simulink model "fft_biplex_real_4x_dsp48_opt_test"  (Simulink 7.4)
settings: Solver=VariableStepDiscrete  StartTime=0.0  StopTime=128  RelTol=1e-3
libraries: xbsIndex_r4 x620, casper_library_misc x24, casper_library_delays x6, casper_library_ffts_twiddle x1, simulink x1
(part 5 of 7)

== system fft_biplex_real_4x_dsp48_opt_test/fft_biplex_real_4x/biplex_core/fft_stage_3/butterfly_direct ==
  a : Inport  OutDataType=sfix(16)  OutScaling=2^0
  b : Inport  Port=2  OutDataType=sfix(16)  OutScaling=2^0
  sync : Inport  Port=3  OutDataType=sfix(16)  OutScaling=2^0
  shift : Inport  Port=4  OutDataType=sfix(16)  OutScaling=2^0
  Logical : xbsIndex_r4/Logical  logical_function=OR  inputs=4  en=off  latency=0  precision=Full  arith_type=Unsigned  n_bits=16  bin_pt=0  align_bp=on  dbl_ovrd=off  block_type=logical
      settings: block_version=11.4
  Mux{0..3} (4 alike) : xbsIndex_r4/Mux  inputs=2  en=off  latency=1  precision=Full  arith_type=Unsigned  n_bits=16  bin_pt=14  quantization=Truncate  overflow=Wrap  dbl_ovrd=off  block_type=mux
      settings: block_version=11.4
  Scale{0..3} (4 alike) : xbsIndex_r4/Scale  scale_factor=-1  dbl_ovrd=off  block_type=scale
  cadd : Subsystem  AncestorBlock=casper_library_misc/caddsub_dsp48e  mask(caddsub_dsp48e){mode=Addition, n_bits_a=8, bin_pt_a=7, n_bits_b=12, bin_pt_b=9, full_precision=on, n_bits_c=19, bin_pt_c=17, quantization=Truncate, overflow=Wrap, cast_latency=0}
      mask prompts: mode "Operation:"; n_bits_a "Bit width 'a':"; bin_pt_a "Binary point 'a':"; n_bits_b "Bit width 'b':"; bin_pt_b "Binary point 'b':"; full_precision "Full precision"; n_bits_c "Bit width out:"; bin_pt_c "Binary point out:"; cast_latency "Cast Latency:"
      mask help:
      | Adds or subtracts two complex numbers using a DSP48E.
      |
      | The two inputs can have different bit widths and binary points, but their sum cannot exceed 24 bits.
      mask init: same as fft_biplex_real_4x_dsp48_opt_test/fft_biplex_real_4x/bi_real_unscr_4x/hilbert_dsp48e0/cadd
      settings: AttributesFormatString=|
      | 8_7 + 12_9 ==> 13_9
      | Mode=Addition
      | Latency=2
      mask StyleString: popup(Addition|Subtraction),edit,edit,edit,edit,checkbox,edit,edit,popup(Truncate|Round  (unbiased: +/- Inf)|Round  (unbiased: Even Values)),popup(Wrap|Saturate|Flag as error),edit
      mask CallbackString:
      | |||||thisVariable = 'full_precision';
      | affectedVars = { ...
      |     'n_bits_c', ...
      |     'bin_pt_c', ...
      |     'quantization', ...
      |     'overflow', ...
      |     'cast_latency', ...
      | };
      | 
      | thisBlock = gcb();
      | thisVarState = get_param(thisBlock, thisVariable);
      | maskNames = get_param(thisBlock, 'MaskNames');
      | maskEnables = get_param(thisBlock, 'MaskEnables');
      | 
      | if strcmp(thisVarState, 'on'),
      |     targVarState = 'off';
      | else,
      |     targVarState = 'on';
      | end
      | 
      | for varName = affectedVars
      |     varIndex = find(ismember(maskNames, varName));
      |     maskEnables{varIndex} = targVarState;
      | end
      | 
      | set_param(thisBlock, 'MaskEnables', maskEnables);|||||
      mask TabNameString: Basic,Basic,Basic,Basic,Basic,Output Type,Output Type,Output Type,Output Type,Output Type,Output Type
  convert_of0 : Subsystem  AncestorBlock=casper_library_misc/convert_of  mask(convert_of){bit_width_i=14, binary_point_i=10, bit_width_o=8, binary_point_o=7, latency=1, overflow=Wrap, quantization=Truncate}
      mask prompts: bit_width_i "Bit Width In"; binary_point_i "Binary Point In"; bit_width_o "Bit Width Out"; binary_point_o "Binary Point Out"; overflow "Overflow Behaviour"; quantization "Quantization Behaviour"
      mask help:
      | Converts from one 2's complement bit-width
      | and/or binary point position to another.
      | Includes underflow/overflow indicator.
      mask init: same as fft_biplex_real_4x_dsp48_opt_test/fft_biplex_real_4x/biplex_core/fft_stage_1/butterfly_direct/convert_of0
      settings: AttributesFormatString=[14,10]->[8,7]
      mask StyleString: edit,edit,edit,edit,edit,popup(Wrap|Saturate|Error),popup(Truncate|Round  (unbiased: +/- Inf)|Round  (unbiased: even values))
  convert_of1 : Subsystem  AncestorBlock=casper_library_misc/convert_of  mask(convert_of){bit_width_i=14, binary_point_i=10, bit_width_o=8, binary_point_o=7, latency=1, overflow=Wrap, quantization=Truncate}
      mask prompts: bit_width_i "Bit Width In"; binary_point_i "Binary Point In"; bit_width_o "Bit Width Out"; binary_point_o "Binary Point Out"; overflow "Overflow Behaviour"; quantization "Quantization Behaviour"
      mask help:
      | Converts from one 2's complement bit-width
      | and/or binary point position to another.
      | Includes underflow/overflow indicator.
      mask init: same as fft_biplex_real_4x_dsp48_opt_test/fft_biplex_real_4x/biplex_core/fft_stage_1/butterfly_direct/convert_of0
      settings: AttributesFormatString=[14,10]->[8,7]
      mask StyleString: edit,edit,edit,edit,edit,popup(Wrap|Saturate|Error),popup(Truncate|Round  (unbiased: +/- Inf)|Round  (unbiased: even values))
  convert_of2 : Subsystem  AncestorBlock=casper_library_misc/convert_of  mask(convert_of){bit_width_i=14, binary_point_i=10, bit_width_o=8, binary_point_o=7, latency=1, overflow=Wrap, quantization=Truncate}
      mask prompts: bit_width_i "Bit Width In"; binary_point_i "Binary Point In"; bit_width_o "Bit Width Out"; binary_point_o "Binary Point Out"; overflow "Overflow Behaviour"; quantization "Quantization Behaviour"
      mask help:
      | Converts from one 2's complement bit-width
      | and/or binary point position to another.
      | Includes underflow/overflow indicator.
      mask init: same as fft_biplex_real_4x_dsp48_opt_test/fft_biplex_real_4x/biplex_core/fft_stage_1/butterfly_direct/convert_of0
      settings: AttributesFormatString=[14,10]->[8,7]
      mask StyleString: edit,edit,edit,edit,edit,popup(Wrap|Saturate|Error),popup(Truncate|Round  (unbiased: +/- Inf)|Round  (unbiased: even values))
  convert_of3 : Subsystem  AncestorBlock=casper_library_misc/convert_of  mask(convert_of){bit_width_i=14, binary_point_i=10, bit_width_o=8, binary_point_o=7, latency=1, overflow=Wrap, quantization=Truncate}
      mask prompts: bit_width_i "Bit Width In"; binary_point_i "Binary Point In"; bit_width_o "Bit Width Out"; binary_point_o "Binary Point Out"; overflow "Overflow Behaviour"; quantization "Quantization Behaviour"
      mask help:
      | Converts from one 2's complement bit-width
      | and/or binary point position to another.
      | Includes underflow/overflow indicator.
      mask init: same as fft_biplex_real_4x_dsp48_opt_test/fft_biplex_real_4x/biplex_core/fft_stage_1/butterfly_direct/convert_of0
      settings: AttributesFormatString=[14,10]->[8,7]
      mask StyleString: edit,edit,edit,edit,edit,popup(Wrap|Saturate|Error),popup(Truncate|Round  (unbiased: +/- Inf)|Round  (unbiased: even values))
  csub : Subsystem  AncestorBlock=casper_library_misc/caddsub_dsp48e  mask(caddsub_dsp48e){mode=Subtraction, n_bits_a=8, bin_pt_a=7, n_bits_b=12, bin_pt_b=9, full_precision=on, n_bits_c=19, bin_pt_c=17, quantization=Truncate, overflow=Wrap, cast_latency=0}
      mask prompts: mode "Operation:"; n_bits_a "Bit width 'a':"; bin_pt_a "Binary point 'a':"; n_bits_b "Bit width 'b':"; bin_pt_b "Binary point 'b':"; full_precision "Full precision"; n_bits_c "Bit width out:"; bin_pt_c "Binary point out:"; cast_latency "Cast Latency:"
      mask help:
      | Adds or subtracts two complex numbers using a DSP48E.
      |
      | The two inputs can have different bit widths and binary points, but their sum cannot exceed 24 bits.
      mask init: same as fft_biplex_real_4x_dsp48_opt_test/fft_biplex_real_4x/bi_real_unscr_4x/hilbert_dsp48e0/cadd
      settings: AttributesFormatString=|
      | 8_7 + 12_9 ==> 13_9
      | Mode=Subtraction
      | Latency=2
      mask StyleString: popup(Addition|Subtraction),edit,edit,edit,edit,checkbox,edit,edit,popup(Truncate|Round  (unbiased: +/- Inf)|Round  (unbiased: Even Values)),popup(Wrap|Saturate|Flag as error),edit
      mask CallbackString:
      | |||||thisVariable = 'full_precision';
      | affectedVars = { ...
      |     'n_bits_c', ...
      |     'bin_pt_c', ...
      |     'quantization', ...
      |     'overflow', ...
      |     'cast_latency', ...
      | };
      | 
      | thisBlock = gcb();
      | thisVarState = get_param(thisBlock, thisVariable);
      | maskNames = get_param(thisBlock, 'MaskNames');
      | maskEnables = get_param(thisBlock, 'MaskEnables');
      | 
      | if strcmp(thisVarState, 'on'),
      |     targVarState = 'off';
      | else,
      |     targVarState = 'on';
      | end
      | 
      | for varName = affectedVars
      |     varIndex = find(ismember(maskNames, varName));
      |     maskEnables{varIndex} = targVarState;
      | end
      | 
      | set_param(thisBlock, 'MaskEnables', maskEnables);|||||
      mask TabNameString: Basic,Basic,Basic,Basic,Basic,Output Type,Output Type,Output Type,Output Type,Output Type,Output Type
  ri_to_c01 : casper_library_misc/ri_to_c  SystemSampleTime=-1
  ri_to_c23 : casper_library_misc/ri_to_c  SystemSampleTime=-1
  shift_delay : xbsIndex_r4/Delay  en=off  latency=2  dbl_ovrd=off  reg_retiming=off  block_type=delay
      settings: block_version=11.4
  sync_delay : xbsIndex_r4/Delay  en=off  latency=4  dbl_ovrd=off  reg_retiming=on  block_type=delay
      settings: block_version=11.4
  twiddle_general_4mult : Subsystem  AncestorBlock=casper_library_ffts_twiddle/twiddle_general_4mult  mask(twiddle_general_4mult){Coeffs=getfield( getfield( get_param( gcb,'UserData' ), 'parameters'),'Coeffs'), StepPeriod=0, coeffs_bram=off, coeff_bit_width=8, input_bit_width=8, add_latency=2, mult_latency=3, bram_latency=1, conv_latency=1, arch=Virtex5, use_hdl=on, use_embedded=off, quantization=Truncate, overflow=Wrap}
      mask prompts: Coeffs "Coefficients:"; StepPeriod "Coefficient Step Period (2^?)"; coeffs_bram "Store coefficients in BRAM"; coeff_bit_width "Coefficient Bit Width"; input_bit_width "Input Bit Width"; add_latency "Add Latency"; mult_latency "Mult Latency"; bram_latency "BRAM Latency"; conv_latency "Convert Latency"; arch "Architecture"; use_hdl "Use behavioural HDL for multipliers"; use_embedded "Use embedded multipliers"; quantization "Quantization Behavior"; overflow "Overflow Behavior"
      mask help:
      | Used in biplex pipelined FFT. Implements
      | (a+bi)(c+di) as (ac-bd)+i(ad+bc) with four
      | multipliers
      mask init:
      | twiddle_general_4mult_init(gcb, ...
      |     'Coeffs', Coeffs, ...
      |     'StepPeriod', StepPeriod, ...
      |     'coeffs_bram', coeffs_bram, ...
      |     'coeff_bit_width', coeff_bit_width, ...
      |     'input_bit_width', input_bit_width, ...
      |     'add_latency', add_latency, ...
      |     'mult_latency', mult_latency, ...
      |     'bram_latency', bram_latency, ...
      |     'conv_latency', conv_latency, ...
      |     'arch', arch, ...
      |     'use_hdl', use_hdl, ...
      |     'use_embedded', use_embedded, ...
      |     'quantization', quantization, ...
      |     'overflow', overflow)
      settings: AttributesFormatString=|
      | data=(8,7)
      | coeffs=(8,6)
      | Virtex5
      | (Truncate,Wrap)
      mask StyleString: edit,edit,checkbox,edit,edit,edit,edit,edit,edit,popup(Virtex2Pro|Virtex5),checkbox,checkbox,popup(Truncate|Round  (unbiased: +/- Inf)|Round  (unbiased: Even Values)),popup(Wrap|Saturate|Error)
      mask CallbackString:
      | ||||||||||use_hdl = get_param(gcb,'use_hdl');
      | visibs = get_param(gcb, 'MaskVisibilities');
      | if( strcmp(use_hdl,'on')),
      |     set_param(gcb, 'use_embedded','off');
      |     visibs{12} = 'off';
      | else,
      |     visibs{12} = 'on';
      | end
      | set_param(gcb, 'MaskVisibilities', visibs);|||
  a+bw : Outport  OutDataType=sfix(16)  OutScaling=2^0
  a-bw : Outport  Port=2  OutDataType=sfix(16)  OutScaling=2^0
  of : Outport  Port=3  OutDataType=sfix(16)  OutScaling=2^0
  sync_out : Outport  Port=4
  wires:
  a/1 -> twiddle_general_4mult/1(a)
  b/1 -> twiddle_general_4mult/2(b)
  sync/1 -> twiddle_general_4mult/3(sync)
  twiddle_general_4mult/1(a_re) -> cadd/1(a_re), csub/1(a_re)
  twiddle_general_4mult/2(a_im) -> cadd/2(a_im), csub/2(a_im)
  twiddle_general_4mult/3(bw_re) -> cadd/3(b_re), csub/3(b_re)
  twiddle_general_4mult/4(bw_im) -> cadd/4(b_im), csub/4(b_im)
  twiddle_general_4mult/5(sync_out) -> sync_delay/1
  shift/1 -> shift_delay/1
  shift_delay/1 -> Mux0/1, Mux1/1, Mux2/1, Mux3/1
  cadd/1(c_re) -> Mux0/2, Scale0/1
  cadd/2(c_im) -> Mux1/2, Scale1/1
  csub/1(c_re) -> Mux2/2, Scale2/1
  csub/2(c_im) -> Mux3/2, Scale3/1
  Scale0/1 -> Mux0/3
  Scale1/1 -> Mux1/3
  Scale2/1 -> Mux2/3
  Scale3/1 -> Mux3/3
  Mux0/1 -> convert_of0/1(din)
  Mux1/1 -> convert_of1/1(din)
  Mux2/1 -> convert_of2/1(din)
  Mux3/1 -> convert_of3/1(din)
  convert_of0/1(dout) -> ri_to_c01/1
  convert_of1/1(dout) -> ri_to_c01/2
  convert_of2/1(dout) -> ri_to_c23/1
  convert_of3/1(dout) -> ri_to_c23/2
  convert_of0/2(of) -> Logical/1
  convert_of1/2(of) -> Logical/2
  convert_of2/2(of) -> Logical/3
  convert_of3/2(of) -> Logical/4
  ri_to_c01/1 -> a+bw/1
  ri_to_c23/1 -> a-bw/1
  Logical/1 -> of/1
  sync_delay/1 -> sync_out/1

== system fft_biplex_real_4x_dsp48_opt_test/fft_biplex_real_4x/biplex_core/fft_stage_3/delay_b ==
  In1 : Inport  OutDataType=sfix(16)  OutScaling=2^0
  delay_slr : xbsIndex_r4/Delay  en=off  latency=DelayLen  dbl_ovrd=off  reg_retiming=off  block_type=delay
      settings: xl_area=[0, 0, 0, 0, 0, 0, 0]  block_version=9.1.01
  Out1 : Outport  OutDataType=sfix(16)  OutScaling=2^0
  wires:
  delay_slr/1 -> Out1/1
  In1/1 -> delay_slr/1

== system fft_biplex_real_4x_dsp48_opt_test/fft_biplex_real_4x/biplex_core/fft_stage_3/delay_f ==
  In1 : Inport  OutDataType=sfix(16)  OutScaling=2^0
  delay_slr : xbsIndex_r4/Delay  en=off  latency=DelayLen  dbl_ovrd=off  reg_retiming=off  block_type=delay
      settings: xl_area=[0, 0, 0, 0, 0, 0, 0]  block_version=9.1.01
  Out1 : Outport  OutDataType=sfix(16)  OutScaling=2^0
  wires:
  delay_slr/1 -> Out1/1
  In1/1 -> delay_slr/1

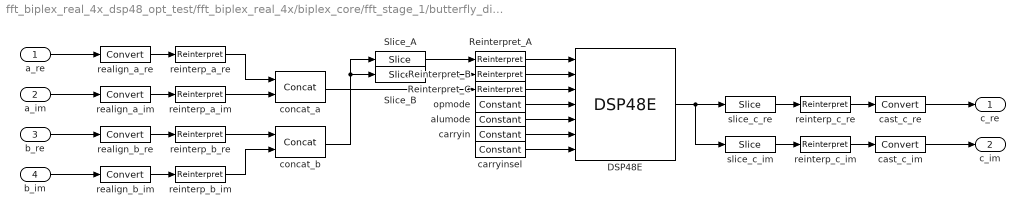
== system fft_biplex_real_4x_dsp48_opt_test/fft_biplex_real_4x/biplex_core/fft_stage_1/butterfly_direct/cadd ==
  a_re : Inport  OutDataType=sfix(16)  OutScaling=2^0
  a_im : Inport  Port=2  OutDataType=sfix(16)  OutScaling=2^0
  b_re : Inport  Port=3  OutDataType=sfix(16)  OutScaling=2^0
  b_im : Inport  Port=4  OutDataType=sfix(16)  OutScaling=2^0
  DSP48E : xbsIndex_r4/DSP48E  use_a=Direct from A Port  use_b=Direct from B Port  pattern_from_creg=off  pattern='000000000000'  mask_from_creg=off  pattern_mask='3FFFFFFFFFFF'  reset_preg=off  sel_rounding_mask=Select mask  use_op=off  use_creg=on  rst_all=off  en_all=off  use_pcin=off  use_carrycascin=off  use_multsignin=off  use_carryout=off  use_patterndetect=off  use_patternbdetect=off  use_overflow=off  use_underflow=off  use_acout=off  use_bcout=off  use_pcout=off  use_multsignout=off  use_carrycascout=off  pipeline_a=1  pipeline_b=1  pipeline_acout=1  pipeline_bcout=1  pipeline_c=on  pipeline_p=on  pipeline_mult=on  pipeline_opmode=on  pipeline_alumode=on  pipeline_carryin=on  pipeline_carryinsel=on  rst_a=off  rst_b=off  rst_c=off  rst_mult=off  rst_p=off  rst_carry_in=off  rst_alumode=off  rst_ctrl=off  en_a1=off  en_a2=off  en_b1=off  en_b2=off  en_c=off  en_mult=off  en_p=off  en_carry_in=off  en_alumode=off  en_multcarryin=off  en_ctrl=off  use_synth_model=off  addsub_mode=TWO24  xl_useadderonly=off  block_type=dsp48e
      settings: block_version=10.1.3
  Reinterpret_A : xbsIndex_r4/Reinterpret  force_arith_type=on  arith_type="Signed  (2's comp)"  force_bin_pt=on  bin_pt=0  block_type=reinterpret
      settings: infoedit="Changes signal type without altering the binary representation.   You can changed the signal between signed and unsigned, and relocate the binary point.<br><br>Hardware notes: In hardware this block costs nothing.<br><br>Example:  Suppose the input is 6 bits wide, signed, with 2 fractional bits, and the output is forced to unsigned with 0 fractional bits.  Then an input of -2.0 (1110.00 in binary 2's complement) becomes an output of 56 (111000 in binary)."  block_version=10.1.3
  Reinterpret_B : xbsIndex_r4/Reinterpret  force_arith_type=on  arith_type="Signed  (2's comp)"  force_bin_pt=on  bin_pt=0  block_type=reinterpret
      settings: infoedit="Changes signal type without altering the binary representation.   You can changed the signal between signed and unsigned, and relocate the binary point.<br><br>Hardware notes: In hardware this block costs nothing.<br><br>Example:  Suppose the input is 6 bits wide, signed, with 2 fractional bits, and the output is forced to unsigned with 0 fractional bits.  Then an input of -2.0 (1110.00 in binary 2's complement) becomes an output of 56 (111000 in binary)."  block_version=10.1.3
  Reinterpret_C : xbsIndex_r4/Reinterpret  force_arith_type=on  arith_type="Signed  (2's comp)"  force_bin_pt=on  bin_pt=0  block_type=reinterpret
      settings: infoedit="Changes signal type without altering the binary representation.   You can changed the signal between signed and unsigned, and relocate the binary point.<br><br>Hardware notes: In hardware this block costs nothing.<br><br>Example:  Suppose the input is 6 bits wide, signed, with 2 fractional bits, and the output is forced to unsigned with 0 fractional bits.  Then an input of -2.0 (1110.00 in binary 2's complement) becomes an output of 56 (111000 in binary)."  block_version=10.1.3
  Slice_A : xbsIndex_r4/Slice  nbits=30  boolean_output=off  mode=Upper Bit Location + Width  bit1=0  base1=MSB of Input  bit0=0  base0=LSB of Input  dbl_ovrd=off  block_type=slice
  Slice_B : xbsIndex_r4/Slice  nbits=18  boolean_output=off  mode=Lower Bit Location + Width  bit1=0  base1=MSB of Input  bit0=0  base0=LSB of Input  dbl_ovrd=off  block_type=slice
  alumode : xbsIndex_r4/Constant  arith_type=Unsigned  const=0  n_bits=4  bin_pt=0  explicit_period=off  period=1  equ=P=C  opselect=C  inp2=PCIN>>17  opr=+  inp1=P  carry=CIN  dbl_ovrd=off  block_type=constant
  carryin : xbsIndex_r4/Constant  arith_type=Unsigned  const=0  n_bits=1  bin_pt=0  explicit_period=off  period=1  equ=P=C  opselect=C  inp2=PCIN>>17  opr=+  inp1=P  carry=CIN  dbl_ovrd=off  block_type=constant
  carryinsel : xbsIndex_r4/Constant  arith_type=Unsigned  const=0  n_bits=3  bin_pt=0  explicit_period=off  period=1  equ=P=C  opselect=C  inp2=PCIN>>17  opr=+  inp1=P  carry=CIN  dbl_ovrd=off  block_type=constant
  cast_c_im : xbsIndex_r4/Convert  arith_type="Signed  (2's comp)"  n_bits=9  bin_pt=7  quantization=Truncate  overflow=Wrap  latency=0  dbl_ovrd=off  pipeline=on  block_type=convert
      settings: block_version=10.1.3
  cast_c_re : xbsIndex_r4/Convert  arith_type="Signed  (2's comp)"  n_bits=9  bin_pt=7  quantization=Truncate  overflow=Wrap  latency=0  dbl_ovrd=off  pipeline=on  block_type=convert
      settings: block_version=10.1.3
  concat_a : xbsIndex_r4/Concat  num_inputs=2  dbl_ovrd=off  block_type=concat
  concat_b : xbsIndex_r4/Concat  num_inputs=2  dbl_ovrd=off  block_type=concat
  opmode : xbsIndex_r4/Constant  arith_type=Unsigned  const=51  n_bits=7  bin_pt=0  explicit_period=off  period=1  equ=P=C  opselect=C  inp2=PCIN>>17  opr=+  inp1=P  carry=CIN  dbl_ovrd=off  block_type=constant
  realign_a_im : xbsIndex_r4/Convert  arith_type="Signed  (2's comp)"  n_bits=24  bin_pt=22  quantization=Truncate  overflow=Wrap  latency=0  dbl_ovrd=off  pipeline=on  block_type=convert
      settings: block_version=10.1.3
  realign_a_re : xbsIndex_r4/Convert  arith_type="Signed  (2's comp)"  n_bits=24  bin_pt=22  quantization=Truncate  overflow=Wrap  latency=0  dbl_ovrd=off  pipeline=on  block_type=convert
      settings: block_version=10.1.3
  realign_b_im : xbsIndex_r4/Convert  arith_type="Signed  (2's comp)"  n_bits=24  bin_pt=22  quantization=Truncate  overflow=Wrap  latency=0  dbl_ovrd=off  pipeline=on  block_type=convert
      settings: block_version=10.1.3
  realign_b_re : xbsIndex_r4/Convert  arith_type="Signed  (2's comp)"  n_bits=24  bin_pt=22  quantization=Truncate  overflow=Wrap  latency=0  dbl_ovrd=off  pipeline=on  block_type=convert
      settings: block_version=10.1.3
  reinterp_a_im : xbsIndex_r4/Reinterpret  force_arith_type=on  arith_type=Unsigned  force_bin_pt=on  bin_pt=0  block_type=reinterpret
      settings: infoedit="Changes signal type without altering the binary representation.   You can changed the signal between signed and unsigned, and relocate the binary point.<br><br>Hardware notes: In hardware this block costs nothing.<br><br>Example:  Suppose the input is 6 bits wide, signed, with 2 fractional bits, and the output is forced to unsigned with 0 fractional bits.  Then an input of -2.0 (1110.00 in binary 2's complement) becomes an output of 56 (111000 in binary)."  block_version=10.1.3
  reinterp_a_re : xbsIndex_r4/Reinterpret  force_arith_type=on  arith_type=Unsigned  force_bin_pt=on  bin_pt=0  block_type=reinterpret
      settings: infoedit="Changes signal type without altering the binary representation.   You can changed the signal between signed and unsigned, and relocate the binary point.<br><br>Hardware notes: In hardware this block costs nothing.<br><br>Example:  Suppose the input is 6 bits wide, signed, with 2 fractional bits, and the output is forced to unsigned with 0 fractional bits.  Then an input of -2.0 (1110.00 in binary 2's complement) becomes an output of 56 (111000 in binary)."  block_version=10.1.3
  reinterp_b_im : xbsIndex_r4/Reinterpret  force_arith_type=on  arith_type=Unsigned  force_bin_pt=on  bin_pt=0  block_type=reinterpret
      settings: infoedit="Changes signal type without altering the binary representation.   You can changed the signal between signed and unsigned, and relocate the binary point.<br><br>Hardware notes: In hardware this block costs nothing.<br><br>Example:  Suppose the input is 6 bits wide, signed, with 2 fractional bits, and the output is forced to unsigned with 0 fractional bits.  Then an input of -2.0 (1110.00 in binary 2's complement) becomes an output of 56 (111000 in binary)."  block_version=10.1.3
  reinterp_b_re : xbsIndex_r4/Reinterpret  force_arith_type=on  arith_type=Unsigned  force_bin_pt=on  bin_pt=0  block_type=reinterpret
      settings: infoedit="Changes signal type without altering the binary representation.   You can changed the signal between signed and unsigned, and relocate the binary point.<br><br>Hardware notes: In hardware this block costs nothing.<br><br>Example:  Suppose the input is 6 bits wide, signed, with 2 fractional bits, and the output is forced to unsigned with 0 fractional bits.  Then an input of -2.0 (1110.00 in binary 2's complement) becomes an output of 56 (111000 in binary)."  block_version=10.1.3
  reinterp_c_im : xbsIndex_r4/Reinterpret  force_arith_type=on  arith_type="Signed  (2's comp)"  force_bin_pt=on  bin_pt=22  block_type=reinterpret
      settings: infoedit="Changes signal type without altering the binary representation.   You can changed the signal between signed and unsigned, and relocate the binary point.<br><br>Hardware notes: In hardware this block costs nothing.<br><br>Example:  Suppose the input is 6 bits wide, signed, with 2 fractional bits, and the output is forced to unsigned with 0 fractional bits.  Then an input of -2.0 (1110.00 in binary 2's complement) becomes an output of 56 (111000 in binary)."  block_version=10.1.3
  reinterp_c_re : xbsIndex_r4/Reinterpret  force_arith_type=on  arith_type="Signed  (2's comp)"  force_bin_pt=on  bin_pt=22  block_type=reinterpret
      settings: infoedit="Changes signal type without altering the binary representation.   You can changed the signal between signed and unsigned, and relocate the binary point.<br><br>Hardware notes: In hardware this block costs nothing.<br><br>Example:  Suppose the input is 6 bits wide, signed, with 2 fractional bits, and the output is forced to unsigned with 0 fractional bits.  Then an input of -2.0 (1110.00 in binary 2's complement) becomes an output of 56 (111000 in binary)."  block_version=10.1.3
  slice_c_im : xbsIndex_r4/Slice  nbits=24  boolean_output=off  mode=Lower Bit Location + Width  bit1=0  base1=MSB of Input  bit0=0  base0=LSB of Input  dbl_ovrd=off  block_type=slice
  slice_c_re : xbsIndex_r4/Slice  nbits=24  boolean_output=off  mode=Lower Bit Location + Width  bit1=0  base1=MSB of Input  bit0=24  base0=LSB of Input  dbl_ovrd=off  block_type=slice
  c_re : Outport  OutDataType=sfix(16)  OutScaling=2^0
  c_im : Outport  Port=2  OutDataType=sfix(16)  OutScaling=2^0
  wires:
  realign_b_im/1 -> reinterp_b_im/1
  realign_b_re/1 -> reinterp_b_re/1
  realign_a_im/1 -> reinterp_a_im/1
  realign_a_re/1 -> reinterp_a_re/1
  a_re/1 -> realign_a_re/1
  b_re/1 -> realign_b_re/1
  Reinterpret_A/1 -> DSP48E/1
  Reinterpret_B/1 -> DSP48E/2
  opmode/1 -> DSP48E/4
  alumode/1 -> DSP48E/5
  carryin/1 -> DSP48E/6
  carryinsel/1 -> DSP48E/7
  a_im/1 -> realign_a_im/1
  b_im/1 -> realign_b_im/1
  concat_a/1 -> Reinterpret_C/1
  Slice_B/1 -> Reinterpret_B/1
  Slice_A/1 -> Reinterpret_A/1
  DSP48E/1 -> slice_c_re/1, slice_c_im/1
  slice_c_re/1 -> reinterp_c_re/1
  slice_c_im/1 -> reinterp_c_im/1
  reinterp_c_re/1 -> cast_c_re/1
  reinterp_c_im/1 -> cast_c_im/1
  Reinterpret_C/1 -> DSP48E/3
  concat_b/1 -> Slice_A/1, Slice_B/1
  reinterp_a_im/1 -> concat_a/2
  reinterp_b_re/1 -> concat_b/1
  reinterp_b_im/1 -> concat_b/2
  reinterp_a_re/1 -> concat_a/1
  cast_c_re/1 -> c_re/1
  cast_c_im/1 -> c_im/1

== system fft_biplex_real_4x_dsp48_opt_test/fft_biplex_real_4x/biplex_core/fft_stage_1/butterfly_direct/convert_of0 ==
  din : Inport  OutDataType=sfix(16)  OutScaling=2^0
  all_0s : xbsIndex_r4/Logical  logical_function=NAND  inputs=2  en=off  latency=latency  precision=Full  arith_type=Unsigned  n_bits=16  bin_pt=0  align_bp=on  dbl_ovrd=off  block_type=logical
  all_1s : xbsIndex_r4/Logical  logical_function=NAND  inputs=2  en=off  latency=latency  precision=Full  arith_type=Unsigned  n_bits=16  bin_pt=0  align_bp=on  dbl_ovrd=off  block_type=logical
  and : xbsIndex_r4/Logical  logical_function=AND  inputs=2  en=off  latency=0  precision=Full  arith_type=Unsigned  n_bits=16  bin_pt=0  align_bp=on  dbl_ovrd=off  block_type=logical
  convert : xbsIndex_r4/Convert  arith_type="Signed  (2's comp)"  n_bits=bit_width_o  bin_pt=binary_point_o  quantization=Truncate  overflow=Wrap  latency=latency  dbl_ovrd=off  pipeline=on  block_type=convert
      settings: block_version=10.1.1
  invert1 : xbsIndex_r4/Inverter  en=off  latency=0  dbl_ovrd=off  block_type=inv
  invert2 : xbsIndex_r4/Inverter  en=off  latency=0  dbl_ovrd=off  block_type=inv
  slice1 : xbsIndex_r4/Slice  nbits=1  boolean_output=on  mode=Upper Bit Location + Width  bit1=0  base1=MSB of Input  bit0=0  base0=LSB of Input  dbl_ovrd=off  block_type=slice
      settings: infoedit="Extracts a given range of bits from each input sample and presents it at the output.  The output type is ordinarily unsigned with binary point at zero, but can be Boolean when the slice is one bit wide.<P><P>Hardware notes: In hardware this block costs nothing."  block_version=10.1.1
  slice2 : xbsIndex_r4/Slice  nbits=1  boolean_output=on  mode=Upper Bit Location + Width  bit1=-1  base1=MSB of Input  bit0=0  base0=LSB of Input  dbl_ovrd=off  block_type=slice
      settings: infoedit="Extracts a given range of bits from each input sample and presents it at the output.  The output type is ordinarily unsigned with binary point at zero, but can be Boolean when the slice is one bit wide.<P><P>Hardware notes: In hardware this block costs nothing."  block_version=10.1.1
  dout : Outport
  of : Outport  Port=2
  wires:
  din/1 -> convert/1, slice1/1, slice2/1
  convert/1 -> dout/1
  slice1/1 -> all_1s/1, invert1/1
  invert1/1 -> all_0s/1
  slice2/1 -> all_1s/2, invert2/1
  invert2/1 -> all_0s/2
  all_0s/1 -> and/1
  all_1s/1 -> and/2
  and/1 -> of/1

== system fft_biplex_real_4x_dsp48_opt_test/fft_biplex_real_4x/biplex_core/fft_stage_1/butterfly_direct/convert_of1 ==
  din : Inport  OutDataType=sfix(16)  OutScaling=2^0
  all_0s : xbsIndex_r4/Logical  logical_function=NAND  inputs=2  en=off  latency=latency  precision=Full  arith_type=Unsigned  n_bits=16  bin_pt=0  align_bp=on  dbl_ovrd=off  block_type=logical
  all_1s : xbsIndex_r4/Logical  logical_function=NAND  inputs=2  en=off  latency=latency  precision=Full  arith_type=Unsigned  n_bits=16  bin_pt=0  align_bp=on  dbl_ovrd=off  block_type=logical
  and : xbsIndex_r4/Logical  logical_function=AND  inputs=2  en=off  latency=0  precision=Full  arith_type=Unsigned  n_bits=16  bin_pt=0  align_bp=on  dbl_ovrd=off  block_type=logical
  convert : xbsIndex_r4/Convert  arith_type="Signed  (2's comp)"  n_bits=bit_width_o  bin_pt=binary_point_o  quantization=Truncate  overflow=Wrap  latency=latency  dbl_ovrd=off  pipeline=on  block_type=convert
      settings: block_version=10.1.1
  invert1 : xbsIndex_r4/Inverter  en=off  latency=0  dbl_ovrd=off  block_type=inv
  invert2 : xbsIndex_r4/Inverter  en=off  latency=0  dbl_ovrd=off  block_type=inv
  slice1 : xbsIndex_r4/Slice  nbits=1  boolean_output=on  mode=Upper Bit Location + Width  bit1=0  base1=MSB of Input  bit0=0  base0=LSB of Input  dbl_ovrd=off  block_type=slice
      settings: infoedit="Extracts a given range of bits from each input sample and presents it at the output.  The output type is ordinarily unsigned with binary point at zero, but can be Boolean when the slice is one bit wide.<P><P>Hardware notes: In hardware this block costs nothing."  block_version=10.1.1
  slice2 : xbsIndex_r4/Slice  nbits=1  boolean_output=on  mode=Upper Bit Location + Width  bit1=-1  base1=MSB of Input  bit0=0  base0=LSB of Input  dbl_ovrd=off  block_type=slice
      settings: infoedit="Extracts a given range of bits from each input sample and presents it at the output.  The output type is ordinarily unsigned with binary point at zero, but can be Boolean when the slice is one bit wide.<P><P>Hardware notes: In hardware this block costs nothing."  block_version=10.1.1
  dout : Outport
  of : Outport  Port=2
  wires:
  din/1 -> convert/1, slice1/1, slice2/1
  convert/1 -> dout/1
  slice1/1 -> all_1s/1, invert1/1
  invert1/1 -> all_0s/1
  slice2/1 -> all_1s/2, invert2/1
  invert2/1 -> all_0s/2
  all_0s/1 -> and/1
  all_1s/1 -> and/2
  and/1 -> of/1

== system fft_biplex_real_4x_dsp48_opt_test/fft_biplex_real_4x/biplex_core/fft_stage_1/butterfly_direct/convert_of2 ==
  din : Inport  OutDataType=sfix(16)  OutScaling=2^0
  all_0s : xbsIndex_r4/Logical  logical_function=NAND  inputs=2  en=off  latency=latency  precision=Full  arith_type=Unsigned  n_bits=16  bin_pt=0  align_bp=on  dbl_ovrd=off  block_type=logical
  all_1s : xbsIndex_r4/Logical  logical_function=NAND  inputs=2  en=off  latency=latency  precision=Full  arith_type=Unsigned  n_bits=16  bin_pt=0  align_bp=on  dbl_ovrd=off  block_type=logical
  and : xbsIndex_r4/Logical  logical_function=AND  inputs=2  en=off  latency=0  precision=Full  arith_type=Unsigned  n_bits=16  bin_pt=0  align_bp=on  dbl_ovrd=off  block_type=logical
  convert : xbsIndex_r4/Convert  arith_type="Signed  (2's comp)"  n_bits=bit_width_o  bin_pt=binary_point_o  quantization=Truncate  overflow=Wrap  latency=latency  dbl_ovrd=off  pipeline=on  block_type=convert
      settings: block_version=10.1.1
  invert1 : xbsIndex_r4/Inverter  en=off  latency=0  dbl_ovrd=off  block_type=inv
  invert2 : xbsIndex_r4/Inverter  en=off  latency=0  dbl_ovrd=off  block_type=inv
  slice1 : xbsIndex_r4/Slice  nbits=1  boolean_output=on  mode=Upper Bit Location + Width  bit1=0  base1=MSB of Input  bit0=0  base0=LSB of Input  dbl_ovrd=off  block_type=slice
      settings: infoedit="Extracts a given range of bits from each input sample and presents it at the output.  The output type is ordinarily unsigned with binary point at zero, but can be Boolean when the slice is one bit wide.<P><P>Hardware notes: In hardware this block costs nothing."  block_version=10.1.1
  slice2 : xbsIndex_r4/Slice  nbits=1  boolean_output=on  mode=Upper Bit Location + Width  bit1=-1  base1=MSB of Input  bit0=0  base0=LSB of Input  dbl_ovrd=off  block_type=slice
      settings: infoedit="Extracts a given range of bits from each input sample and presents it at the output.  The output type is ordinarily unsigned with binary point at zero, but can be Boolean when the slice is one bit wide.<P><P>Hardware notes: In hardware this block costs nothing."  block_version=10.1.1
  dout : Outport
  of : Outport  Port=2
  wires:
  din/1 -> convert/1, slice1/1, slice2/1
  convert/1 -> dout/1
  slice1/1 -> all_1s/1, invert1/1
  invert1/1 -> all_0s/1
  slice2/1 -> all_1s/2, invert2/1
  invert2/1 -> all_0s/2
  all_0s/1 -> and/1
  all_1s/1 -> and/2
  and/1 -> of/1

== system fft_biplex_real_4x_dsp48_opt_test/fft_biplex_real_4x/biplex_core/fft_stage_1/butterfly_direct/convert_of3 ==
  din : Inport  OutDataType=sfix(16)  OutScaling=2^0
  all_0s : xbsIndex_r4/Logical  logical_function=NAND  inputs=2  en=off  latency=latency  precision=Full  arith_type=Unsigned  n_bits=16  bin_pt=0  align_bp=on  dbl_ovrd=off  block_type=logical
  all_1s : xbsIndex_r4/Logical  logical_function=NAND  inputs=2  en=off  latency=latency  precision=Full  arith_type=Unsigned  n_bits=16  bin_pt=0  align_bp=on  dbl_ovrd=off  block_type=logical
  and : xbsIndex_r4/Logical  logical_function=AND  inputs=2  en=off  latency=0  precision=Full  arith_type=Unsigned  n_bits=16  bin_pt=0  align_bp=on  dbl_ovrd=off  block_type=logical
  convert : xbsIndex_r4/Convert  arith_type="Signed  (2's comp)"  n_bits=bit_width_o  bin_pt=binary_point_o  quantization=Truncate  overflow=Wrap  latency=latency  dbl_ovrd=off  pipeline=on  block_type=convert
      settings: block_version=10.1.1
  invert1 : xbsIndex_r4/Inverter  en=off  latency=0  dbl_ovrd=off  block_type=inv
  invert2 : xbsIndex_r4/Inverter  en=off  latency=0  dbl_ovrd=off  block_type=inv
  slice1 : xbsIndex_r4/Slice  nbits=1  boolean_output=on  mode=Upper Bit Location + Width  bit1=0  base1=MSB of Input  bit0=0  base0=LSB of Input  dbl_ovrd=off  block_type=slice
      settings: infoedit="Extracts a given range of bits from each input sample and presents it at the output.  The output type is ordinarily unsigned with binary point at zero, but can be Boolean when the slice is one bit wide.<P><P>Hardware notes: In hardware this block costs nothing."  block_version=10.1.1
  slice2 : xbsIndex_r4/Slice  nbits=1  boolean_output=on  mode=Upper Bit Location + Width  bit1=-1  base1=MSB of Input  bit0=0  base0=LSB of Input  dbl_ovrd=off  block_type=slice
      settings: infoedit="Extracts a given range of bits from each input sample and presents it at the output.  The output type is ordinarily unsigned with binary point at zero, but can be Boolean when the slice is one bit wide.<P><P>Hardware notes: In hardware this block costs nothing."  block_version=10.1.1
  dout : Outport
  of : Outport  Port=2
  wires:
  din/1 -> convert/1, slice1/1, slice2/1
  convert/1 -> dout/1
  slice1/1 -> all_1s/1, invert1/1
  invert1/1 -> all_0s/1
  slice2/1 -> all_1s/2, invert2/1
  invert2/1 -> all_0s/2
  all_0s/1 -> and/1
  all_1s/1 -> and/2
  and/1 -> of/1

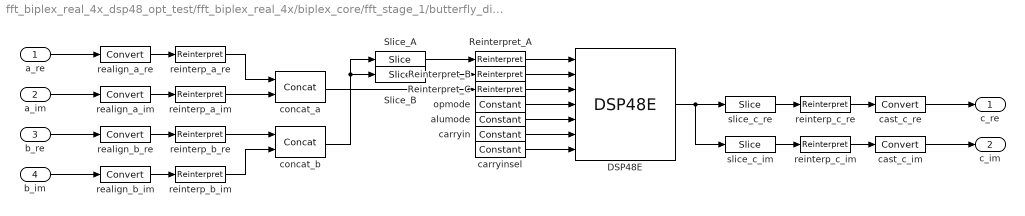
== system fft_biplex_real_4x_dsp48_opt_test/fft_biplex_real_4x/biplex_core/fft_stage_1/butterfly_direct/csub ==
  a_re : Inport  OutDataType=sfix(16)  OutScaling=2^0
  a_im : Inport  Port=2  OutDataType=sfix(16)  OutScaling=2^0
  b_re : Inport  Port=3  OutDataType=sfix(16)  OutScaling=2^0
  b_im : Inport  Port=4  OutDataType=sfix(16)  OutScaling=2^0
  DSP48E : xbsIndex_r4/DSP48E  use_a=Direct from A Port  use_b=Direct from B Port  pattern_from_creg=off  pattern='000000000000'  mask_from_creg=off  pattern_mask='3FFFFFFFFFFF'  reset_preg=off  sel_rounding_mask=Select mask  use_op=off  use_creg=on  rst_all=off  en_all=off  use_pcin=off  use_carrycascin=off  use_multsignin=off  use_carryout=off  use_patterndetect=off  use_patternbdetect=off  use_overflow=off  use_underflow=off  use_acout=off  use_bcout=off  use_pcout=off  use_multsignout=off  use_carrycascout=off  pipeline_a=1  pipeline_b=1  pipeline_acout=1  pipeline_bcout=1  pipeline_c=on  pipeline_p=on  pipeline_mult=on  pipeline_opmode=on  pipeline_alumode=on  pipeline_carryin=on  pipeline_carryinsel=on  rst_a=off  rst_b=off  rst_c=off  rst_mult=off  rst_p=off  rst_carry_in=off  rst_alumode=off  rst_ctrl=off  en_a1=off  en_a2=off  en_b1=off  en_b2=off  en_c=off  en_mult=off  en_p=off  en_carry_in=off  en_alumode=off  en_multcarryin=off  en_ctrl=off  use_synth_model=off  addsub_mode=TWO24  xl_useadderonly=off  block_type=dsp48e
      settings: block_version=10.1.3
  Reinterpret_A : xbsIndex_r4/Reinterpret  force_arith_type=on  arith_type="Signed  (2's comp)"  force_bin_pt=on  bin_pt=0  block_type=reinterpret
      settings: infoedit="Changes signal type without altering the binary representation.   You can changed the signal between signed and unsigned, and relocate the binary point.<br><br>Hardware notes: In hardware this block costs nothing.<br><br>Example:  Suppose the input is 6 bits wide, signed, with 2 fractional bits, and the output is forced to unsigned with 0 fractional bits.  Then an input of -2.0 (1110.00 in binary 2's complement) becomes an output of 56 (111000 in binary)."  block_version=10.1.3
  Reinterpret_B : xbsIndex_r4/Reinterpret  force_arith_type=on  arith_type="Signed  (2's comp)"  force_bin_pt=on  bin_pt=0  block_type=reinterpret
      settings: infoedit="Changes signal type without altering the binary representation.   You can changed the signal between signed and unsigned, and relocate the binary point.<br><br>Hardware notes: In hardware this block costs nothing.<br><br>Example:  Suppose the input is 6 bits wide, signed, with 2 fractional bits, and the output is forced to unsigned with 0 fractional bits.  Then an input of -2.0 (1110.00 in binary 2's complement) becomes an output of 56 (111000 in binary)."  block_version=10.1.3
  Reinterpret_C : xbsIndex_r4/Reinterpret  force_arith_type=on  arith_type="Signed  (2's comp)"  force_bin_pt=on  bin_pt=0  block_type=reinterpret
      settings: infoedit="Changes signal type without altering the binary representation.   You can changed the signal between signed and unsigned, and relocate the binary point.<br><br>Hardware notes: In hardware this block costs nothing.<br><br>Example:  Suppose the input is 6 bits wide, signed, with 2 fractional bits, and the output is forced to unsigned with 0 fractional bits.  Then an input of -2.0 (1110.00 in binary 2's complement) becomes an output of 56 (111000 in binary)."  block_version=10.1.3
  Slice_A : xbsIndex_r4/Slice  nbits=30  boolean_output=off  mode=Upper Bit Location + Width  bit1=0  base1=MSB of Input  bit0=0  base0=LSB of Input  dbl_ovrd=off  block_type=slice
  Slice_B : xbsIndex_r4/Slice  nbits=18  boolean_output=off  mode=Lower Bit Location + Width  bit1=0  base1=MSB of Input  bit0=0  base0=LSB of Input  dbl_ovrd=off  block_type=slice
  alumode : xbsIndex_r4/Constant  arith_type=Unsigned  const=3  n_bits=4  bin_pt=0  explicit_period=off  period=1  equ=P=C  opselect=C  inp2=PCIN>>17  opr=+  inp1=P  carry=CIN  dbl_ovrd=off  block_type=constant
  carryin : xbsIndex_r4/Constant  arith_type=Unsigned  const=0  n_bits=1  bin_pt=0  explicit_period=off  period=1  equ=P=C  opselect=C  inp2=PCIN>>17  opr=+  inp1=P  carry=CIN  dbl_ovrd=off  block_type=constant
  carryinsel : xbsIndex_r4/Constant  arith_type=Unsigned  const=0  n_bits=3  bin_pt=0  explicit_period=off  period=1  equ=P=C  opselect=C  inp2=PCIN>>17  opr=+  inp1=P  carry=CIN  dbl_ovrd=off  block_type=constant
  cast_c_im : xbsIndex_r4/Convert  arith_type="Signed  (2's comp)"  n_bits=9  bin_pt=7  quantization=Truncate  overflow=Wrap  latency=0  dbl_ovrd=off  pipeline=on  block_type=convert
      settings: block_version=10.1.3
  cast_c_re : xbsIndex_r4/Convert  arith_type="Signed  (2's comp)"  n_bits=9  bin_pt=7  quantization=Truncate  overflow=Wrap  latency=0  dbl_ovrd=off  pipeline=on  block_type=convert
      settings: block_version=10.1.3
  concat_a : xbsIndex_r4/Concat  num_inputs=2  dbl_ovrd=off  block_type=concat
  concat_b : xbsIndex_r4/Concat  num_inputs=2  dbl_ovrd=off  block_type=concat
  opmode : xbsIndex_r4/Constant  arith_type=Unsigned  const=51  n_bits=7  bin_pt=0  explicit_period=off  period=1  equ=P=C  opselect=C  inp2=PCIN>>17  opr=+  inp1=P  carry=CIN  dbl_ovrd=off  block_type=constant
  realign_a_im : xbsIndex_r4/Convert  arith_type="Signed  (2's comp)"  n_bits=24  bin_pt=22  quantization=Truncate  overflow=Wrap  latency=0  dbl_ovrd=off  pipeline=on  block_type=convert
      settings: block_version=10.1.3
  realign_a_re : xbsIndex_r4/Convert  arith_type="Signed  (2's comp)"  n_bits=24  bin_pt=22  quantization=Truncate  overflow=Wrap  latency=0  dbl_ovrd=off  pipeline=on  block_type=convert
      settings: block_version=10.1.3
  realign_b_im : xbsIndex_r4/Convert  arith_type="Signed  (2's comp)"  n_bits=24  bin_pt=22  quantization=Truncate  overflow=Wrap  latency=0  dbl_ovrd=off  pipeline=on  block_type=convert
      settings: block_version=10.1.3
  realign_b_re : xbsIndex_r4/Convert  arith_type="Signed  (2's comp)"  n_bits=24  bin_pt=22  quantization=Truncate  overflow=Wrap  latency=0  dbl_ovrd=off  pipeline=on  block_type=convert
      settings: block_version=10.1.3
  reinterp_a_im : xbsIndex_r4/Reinterpret  force_arith_type=on  arith_type=Unsigned  force_bin_pt=on  bin_pt=0  block_type=reinterpret
      settings: infoedit="Changes signal type without altering the binary representation.   You can changed the signal between signed and unsigned, and relocate the binary point.<br><br>Hardware notes: In hardware this block costs nothing.<br><br>Example:  Suppose the input is 6 bits wide, signed, with 2 fractional bits, and the output is forced to unsigned with 0 fractional bits.  Then an input of -2.0 (1110.00 in binary 2's complement) becomes an output of 56 (111000 in binary)."  block_version=10.1.3
  reinterp_a_re : xbsIndex_r4/Reinterpret  force_arith_type=on  arith_type=Unsigned  force_bin_pt=on  bin_pt=0  block_type=reinterpret
      settings: infoedit="Changes signal type without altering the binary representation.   You can changed the signal between signed and unsigned, and relocate the binary point.<br><br>Hardware notes: In hardware this block costs nothing.<br><br>Example:  Suppose the input is 6 bits wide, signed, with 2 fractional bits, and the output is forced to unsigned with 0 fractional bits.  Then an input of -2.0 (1110.00 in binary 2's complement) becomes an output of 56 (111000 in binary)."  block_version=10.1.3
  reinterp_b_im : xbsIndex_r4/Reinterpret  force_arith_type=on  arith_type=Unsigned  force_bin_pt=on  bin_pt=0  block_type=reinterpret
      settings: infoedit="Changes signal type without altering the binary representation.   You can changed the signal between signed and unsigned, and relocate the binary point.<br><br>Hardware notes: In hardware this block costs nothing.<br><br>Example:  Suppose the input is 6 bits wide, signed, with 2 fractional bits, and the output is forced to unsigned with 0 fractional bits.  Then an input of -2.0 (1110.00 in binary 2's complement) becomes an output of 56 (111000 in binary)."  block_version=10.1.3
  reinterp_b_re : xbsIndex_r4/Reinterpret  force_arith_type=on  arith_type=Unsigned  force_bin_pt=on  bin_pt=0  block_type=reinterpret
      settings: infoedit="Changes signal type without altering the binary representation.   You can changed the signal between signed and unsigned, and relocate the binary point.<br><br>Hardware notes: In hardware this block costs nothing.<br><br>Example:  Suppose the input is 6 bits wide, signed, with 2 fractional bits, and the output is forced to unsigned with 0 fractional bits.  Then an input of -2.0 (1110.00 in binary 2's complement) becomes an output of 56 (111000 in binary)."  block_version=10.1.3
  reinterp_c_im : xbsIndex_r4/Reinterpret  force_arith_type=on  arith_type="Signed  (2's comp)"  force_bin_pt=on  bin_pt=22  block_type=reinterpret
      settings: infoedit="Changes signal type without altering the binary representation.   You can changed the signal between signed and unsigned, and relocate the binary point.<br><br>Hardware notes: In hardware this block costs nothing.<br><br>Example:  Suppose the input is 6 bits wide, signed, with 2 fractional bits, and the output is forced to unsigned with 0 fractional bits.  Then an input of -2.0 (1110.00 in binary 2's complement) becomes an output of 56 (111000 in binary)."  block_version=10.1.3
  reinterp_c_re : xbsIndex_r4/Reinterpret  force_arith_type=on  arith_type="Signed  (2's comp)"  force_bin_pt=on  bin_pt=22  block_type=reinterpret
      settings: infoedit="Changes signal type without altering the binary representation.   You can changed the signal between signed and unsigned, and relocate the binary point.<br><br>Hardware notes: In hardware this block costs nothing.<br><br>Example:  Suppose the input is 6 bits wide, signed, with 2 fractional bits, and the output is forced to unsigned with 0 fractional bits.  Then an input of -2.0 (1110.00 in binary 2's complement) becomes an output of 56 (111000 in binary)."  block_version=10.1.3
  slice_c_im : xbsIndex_r4/Slice  nbits=24  boolean_output=off  mode=Lower Bit Location + Width  bit1=0  base1=MSB of Input  bit0=0  base0=LSB of Input  dbl_ovrd=off  block_type=slice
  slice_c_re : xbsIndex_r4/Slice  nbits=24  boolean_output=off  mode=Lower Bit Location + Width  bit1=0  base1=MSB of Input  bit0=24  base0=LSB of Input  dbl_ovrd=off  block_type=slice
  c_re : Outport  OutDataType=sfix(16)  OutScaling=2^0
  c_im : Outport  Port=2  OutDataType=sfix(16)  OutScaling=2^0
  wires:
  realign_b_im/1 -> reinterp_b_im/1
  realign_b_re/1 -> reinterp_b_re/1
  realign_a_im/1 -> reinterp_a_im/1
  realign_a_re/1 -> reinterp_a_re/1
  a_re/1 -> realign_a_re/1
  b_re/1 -> realign_b_re/1
  Reinterpret_A/1 -> DSP48E/1
  Reinterpret_B/1 -> DSP48E/2
  opmode/1 -> DSP48E/4
  alumode/1 -> DSP48E/5
  carryin/1 -> DSP48E/6
  carryinsel/1 -> DSP48E/7
  a_im/1 -> realign_a_im/1
  b_im/1 -> realign_b_im/1
  concat_a/1 -> Reinterpret_C/1
  Slice_B/1 -> Reinterpret_B/1
  Slice_A/1 -> Reinterpret_A/1
  DSP48E/1 -> slice_c_re/1, slice_c_im/1
  slice_c_re/1 -> reinterp_c_re/1
  slice_c_im/1 -> reinterp_c_im/1
  reinterp_c_re/1 -> cast_c_re/1
  reinterp_c_im/1 -> cast_c_im/1
  Reinterpret_C/1 -> DSP48E/3
  concat_b/1 -> Slice_A/1, Slice_B/1
  reinterp_a_im/1 -> concat_a/2
  reinterp_b_re/1 -> concat_b/1
  reinterp_b_im/1 -> concat_b/2
  reinterp_a_re/1 -> concat_a/1
  cast_c_re/1 -> c_re/1
  cast_c_im/1 -> c_im/1
